simulink library "Engine_Lib"  (R2025a)
settings: Solver=ode45  StartTime=0.0  StopTime=10.0  RelTol=1e-3  EnableMultiTasking=on
undefined symbols (not defined in the file or in its folder): AFR_Table, beta, center, coeffs, DCT_Param, ECP_Table, exponent, ICP_Table, invDG, Load_Table, numterms, polyTerms, S_Table, WendlandNumTerms, width
libraries: fl_lib x8, nesl_utility x6, sdl_lib x1
(part 2 of 2)

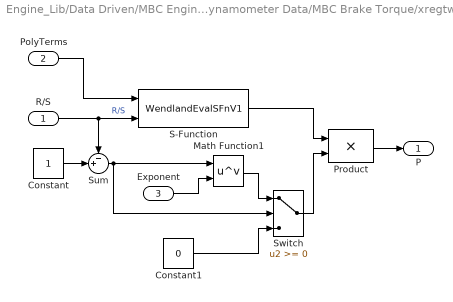
== system Engine_Lib/Data Driven/MBC Engine Model From Dynamometer Data/MBC Brake Torque/xregtwostage/RF1/hybridRBFEval/rbfwendlandEval/Wendland ==
  R/S : Inport
  PolyTerms : Inport  Port=2
  Exponent : Inport  Port=3
  Constant : Constant
  Constant1 : Constant  Value=0
  Math Function1 : Math  Operator=pow  SignedPower=on
  Product : Product  InputSameDT=on  SaturateOnIntegerOverflow=on  OutDataTypeStr=Inherit: Same as first input
  S-Function : S-Function  FunctionName=WendlandEvalSFnV1  Parameters=NumTerms  SFunctionDeploymentMode=off  EnableBusSupport=off
  Sum : Sum  Inputs=-+|  InputSameDT=on  SaturateOnIntegerOverflow=on  OutDataTypeStr=Inherit: Same as first input
  Switch : Switch  SaturateOnIntegerOverflow=off
  P : Outport  VectorParamsAs1DForOutWhenUnconnected=off
  wires:
  Product/1 -> P/1
  R/S/1 -> S-Function/2, Sum/1  "R/S"
  PolyTerms/1 -> S-Function/1
  Constant/1 -> Sum/2
  Exponent/1 -> Math Function1/2
  Constant1/1 -> Switch/3
  S-Function/1 -> Product/1
  Sum/1 -> Math Function1/1, Switch/2
  Math Function1/1 -> Switch/1
  Switch/1 -> Product/2

== system Engine_Lib/Data Driven/MBC Engine Model From Dynamometer Data/MBC Brake Torque/xregtwostage/RF2/hybridRBFEval/rbfmultiquadricEval/MqGlobalWidth ==
  note: If Sigma has more than one width per dimension
      | then y = sqrt ((R/S)^2 +1)
      | otherwise y = S * sqrt ((R/S)^2 +1)
      |
      | This subsystem deals with the global width case.
      | See Multiquadric for thewidth/dim, width/center
      | and width/center/dim cases.
  (R/S)^2 : Inport
  S : Inport  Port=2
  Constant1 : Constant
  Math Function2 : Math  Operator=sqrt  SignedPower=on
  Product : Product  InputSameDT=on  SaturateOnIntegerOverflow=on  OutDataTypeStr=Inherit: Same as first input
  Selector : Selector  NumberOfDimensions=2  IndexOptions=Index vector (dialog),Index vector (dialog)  Indices=1,1  OutputSizes=1
  Sum : Sum  Inputs=++|  InputSameDT=on  SaturateOnIntegerOverflow=on  OutDataTypeStr=Inherit: Same as first input
  P : Outport  VectorParamsAs1DForOutWhenUnconnected=off
  wires:
  Selector/1 -> Product/2
  Product/1 -> P/1
  Math Function2/1 -> Product/1
  Constant1/1 -> Sum/1
  (R/S)^2/1 -> Sum/2
  Sum/1 -> Math Function2/1
  S/1 -> Selector/1

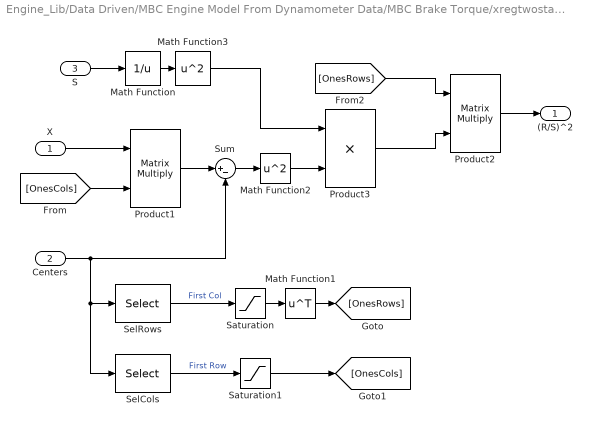
== system Engine_Lib/Data Driven/MBC Engine Model From Dynamometer Data/MBC Brake Torque/xregtwostage/RF2/hybridRBFEval/rbfmultiquadricEval/R ==
  X : Inport
  "Centers " : Inport  Port=2
  S : Inport  Port=3
  Math Function : Math  Operator=reciprocal  SignedPower=on
  Math Function1 : Math  Operator=transpose  SignedPower=on
  Math Function2 : Math  Operator=square  SignedPower=on
  Math Function3 : Math  Operator=square  SignedPower=on
  Product1 : Product  Multiplication=Matrix(*)  InputSameDT=on  SaturateOnIntegerOverflow=on  OutDataTypeStr=Inherit: Same as first input
  Product2 : Product  Multiplication=Matrix(*)  InputSameDT=on  SaturateOnIntegerOverflow=on  OutDataTypeStr=Inherit: Same as first input
  Product3 : Product  InputSameDT=on  SaturateOnIntegerOverflow=on  OutDataTypeStr=Inherit: Same as first input
  Saturation : Saturate  UpperLimit=1  LowerLimit=1
  Saturation1 : Saturate  UpperLimit=1  LowerLimit=1
  SelCols : Selector  NumberOfDimensions=2  InputPortWidth=3  IndexOptions=Index vector (dialog),Select all  Indices=1,-1  OutputSizes=1
  SelRows : Selector  NumberOfDimensions=2  InputPortWidth=3  IndexOptions=Select all,Index vector (dialog)  Indices=-1,1  OutputSizes=1
  Sum : Sum  Inputs=|+-  InputSameDT=on  SaturateOnIntegerOverflow=on  OutDataTypeStr=Inherit: Same as first input
  (R/S)^2 : Outport  VectorParamsAs1DForOutWhenUnconnected=off
  wires:
  Math Function2/1 -> Product3/2
  Sum/1 -> Math Function2/1
  Product1/1 -> Sum/1
  X/1 -> Product1/1
  [OnesCols] -> Product1/2
  Math Function1/1 -> [OnesRows]
  SelRows/1 -> Saturation/1  "First Col"
  "Centers "/1 -> Sum/2, SelRows/1, SelCols/1
  S/1 -> Math Function/1
  Math Function/1 -> Math Function3/1
  Saturation/1 -> Math Function1/1
  SelCols/1 -> Saturation1/1  "First Row"
  Saturation1/1 -> [OnesCols]
  Math Function3/1 -> Product3/1
  Product3/1 -> Product2/2
  Product2/1 -> (R/S)^2/1
  [OnesRows] -> Product2/1

== system Engine_Lib/Data Driven/MBC Engine Model From Dynamometer Data/MBC Brake Torque/xregtwostage/RF3/hybridRBFEval/rbfmultiquadricEval/MqGlobalWidth ==
  note: If Sigma has more than one width per dimension
      | then y = sqrt ((R/S)^2 +1)
      | otherwise y = S * sqrt ((R/S)^2 +1)
      |
      | This subsystem deals with the global width case.
      | See Multiquadric for thewidth/dim, width/center
      | and width/center/dim cases.
  (R/S)^2 : Inport
  S : Inport  Port=2
  Constant1 : Constant
  Math Function2 : Math  Operator=sqrt  SignedPower=on
  Product : Product  InputSameDT=on  SaturateOnIntegerOverflow=on  OutDataTypeStr=Inherit: Same as first input
  Selector : Selector  NumberOfDimensions=2  IndexOptions=Index vector (dialog),Index vector (dialog)  Indices=1,1  OutputSizes=1
  Sum : Sum  Inputs=++|  InputSameDT=on  SaturateOnIntegerOverflow=on  OutDataTypeStr=Inherit: Same as first input
  P : Outport  VectorParamsAs1DForOutWhenUnconnected=off
  wires:
  Selector/1 -> Product/2
  Product/1 -> P/1
  Math Function2/1 -> Product/1
  Constant1/1 -> Sum/1
  (R/S)^2/1 -> Sum/2
  Sum/1 -> Math Function2/1
  S/1 -> Selector/1

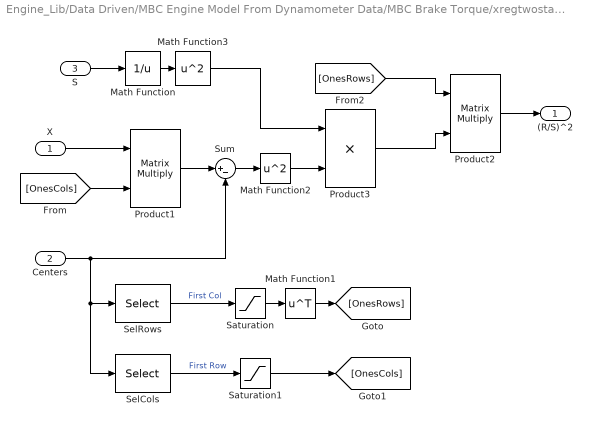
== system Engine_Lib/Data Driven/MBC Engine Model From Dynamometer Data/MBC Brake Torque/xregtwostage/RF3/hybridRBFEval/rbfmultiquadricEval/R ==
  X : Inport
  "Centers " : Inport  Port=2
  S : Inport  Port=3
  Math Function : Math  Operator=reciprocal  SignedPower=on
  Math Function1 : Math  Operator=transpose  SignedPower=on
  Math Function2 : Math  Operator=square  SignedPower=on
  Math Function3 : Math  Operator=square  SignedPower=on
  Product1 : Product  Multiplication=Matrix(*)  InputSameDT=on  SaturateOnIntegerOverflow=on  OutDataTypeStr=Inherit: Same as first input
  Product2 : Product  Multiplication=Matrix(*)  InputSameDT=on  SaturateOnIntegerOverflow=on  OutDataTypeStr=Inherit: Same as first input
  Product3 : Product  InputSameDT=on  SaturateOnIntegerOverflow=on  OutDataTypeStr=Inherit: Same as first input
  Saturation : Saturate  UpperLimit=1  LowerLimit=1
  Saturation1 : Saturate  UpperLimit=1  LowerLimit=1
  SelCols : Selector  NumberOfDimensions=2  InputPortWidth=3  IndexOptions=Index vector (dialog),Select all  Indices=1,-1  OutputSizes=1
  SelRows : Selector  NumberOfDimensions=2  InputPortWidth=3  IndexOptions=Select all,Index vector (dialog)  Indices=-1,1  OutputSizes=1
  Sum : Sum  Inputs=|+-  InputSameDT=on  SaturateOnIntegerOverflow=on  OutDataTypeStr=Inherit: Same as first input
  (R/S)^2 : Outport  VectorParamsAs1DForOutWhenUnconnected=off
  wires:
  Math Function2/1 -> Product3/2
  Sum/1 -> Math Function2/1
  Product1/1 -> Sum/1
  X/1 -> Product1/1
  [OnesCols] -> Product1/2
  Math Function1/1 -> [OnesRows]
  SelRows/1 -> Saturation/1  "First Col"
  "Centers "/1 -> Sum/2, SelRows/1, SelCols/1
  S/1 -> Math Function/1
  Math Function/1 -> Math Function3/1
  Saturation/1 -> Math Function1/1
  SelCols/1 -> Saturation1/1  "First Row"
  Saturation1/1 -> [OnesCols]
  Math Function3/1 -> Product3/1
  Product3/1 -> Product2/2
  Product2/1 -> (R/S)^2/1
  [OnesRows] -> Product2/1
